simulink model "OSWEC_Hydraulic_PTO"  (R2020b)
settings: Solver=ode4  StartTime=0  StopTime=400  FixedStep=0.01  MaxStep=0.01  RelTol=1e-3  EnableMultiTasking=on
undefined symbols (not defined in the file or in its folder): body, constraint, geometry, hydroData, pto, PTOControl, ptoSim
libraries: WECSim_Lib_PTOSim x7, WECSim_Lib_Body_Elements x2, WECSim_Lib_Constraints x1, WECSim_Lib_Frames x1, pid_lib x1, WECSim_Lib_PTOs x1
settings Model: Creator=mlawson  LastModifiedBy=jleonqu
settings SolverCC: ZeroCrossControl=DisableAll  AlgebraicLoopSolver=LineSearch  AutoInsertRateTranBlk=on
settings DataIOCC: SaveFormat=Array  SaveOutput=off  SaveTime=off  ReturnWorkspaceOutputs=off
settings OptimizationCC: LifeSpan=inf  SimCompilerOptimization=on
settings DebuggingCC: UnderspecifiedInitializationDetection=Classic  MergeDetectMultiDrivingBlocksExec=none  SolverPrmCheckMsg=warning  AllowSymbolicDim=off  StateNameClashWarn=warning  SFUnexpectedBacktrackingDiag=warning  SFNoUnconditionalDefaultTransitionDiag=warning  ArithmeticOperatorsInVariantConditions=warning
settings HardwareCC: ProdBitPerPointer=32  ProdBitPerSizeT=32  ProdBitPerPtrDiffT=32  ProdLargestAtomicFloat=None  ProdIntDivRoundTo=Undefined  ProdEndianess=Unspecified  ProdWordSize=32  ProdHWDeviceType=32-bit Generic
settings ModelReferenceCC: PropagateSignalLabelsOutOfModel=off
settings SFSimCC: SimUseLocalCustomCode=off  CustomCodeUndefinedFunction=UseInterfaceOnly
settings RTWCC: RTWUseLocalCustomCode=off
settings CodeAppCC: StateflowObjectComments=on
settings GRTTargetCC: TargetLangStandard=C89/C90 (ANSI)
settings ConfigComp: CovMetricSettings=dw  CovSaveCumulativeToWorkspaceVar=on  CovSaveSingleToWorkspaceVar=on  CovExternalEMLEnable=off  CovSFcnEnable=off
settings SimscapeCC: SimscapeNormalizeSystem=off
settings ConfigurationSet: Description=SimMechanics 2G
settings ExplorerConfigSet: SimMechanicsOpenEditorOnUpdate=off  InternalSimMechanicsExplorerSettings="<ExplorerConfiguration><canonicalview>default</canonicalview><TilePanel><TileInfo><Tiles Columns=\"1\" Count=\"1\" Rows=\"1\"><Column Left=\"2\" Weight=\"1\"/><Column Left=\"1335\"/><Row Top=\"2\" Weight=\"1\"/><Row Top=\"911\"/><Tile Height=\"1\" Width=\"1\" X=\"0\" Y=\"0\"/></Tiles></TileInfo><SceneInfo><SceneViewer><BGColor><R>0.60000002384185791</R><G>0.60000002384185791</G><B>0.60000002384185791</B></BGColor><Camera><Position><X>365.37645888990272</X><Y>-369.82486814446582</Y><Z>359.64809521743916</Z></Position><Center><X>-6.7351450971904585</X><Y>2.2867358426280204</Y><Z>-12.463508769654169</Z></Center><Up><X>-0.40824829046386307</X><Y>0.40824829046386307</Y><Z>0.81649658092772615</Z></Up><Left>-57.820127362122818</Left><Right>57.820127362122818</Right><Bottom>-38.308817187253304</Bottom><Top>38.308817187253304</Top></Camera></SceneViewer></SceneInfo></TilePanel></ExplorerConfiguration>"

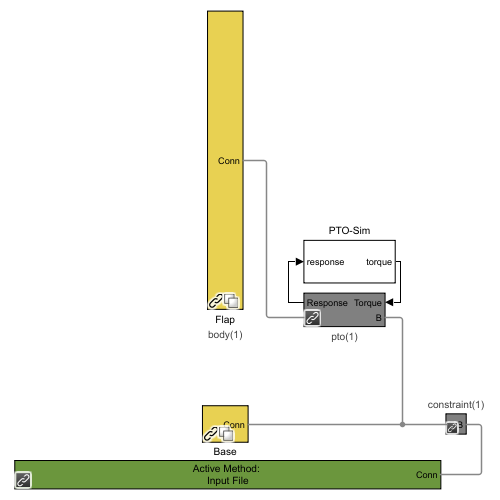
[thumbnail: Simulink's stored preview of the top-level diagram]
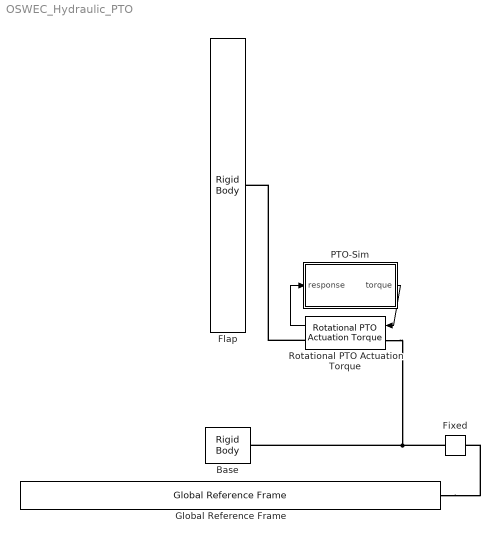
== system OSWEC_Hydraulic_PTO ==
  Base : WECSim_Lib_Body_Elements/Rigid Body  body=body(2)  h5File=hydroData/*.h5  geometryFile=geometry/*.stl  mass=0  inertia=0 0 0  inertiaProducts=0 0 0  nonHydro=0  nonlinearHydro=0  centerGravity=0 0 0  centerBuoyancy=0 0 0  dof=6  volume=0  displacement=0 0 0  axis=0 1 0  angle=0  option=0  cd=0 0 0  ca=0 0 0  area=0 0 0  VME=0  rgME=0 0 0  z=0 0 1
  Fixed : WECSim_Lib_Constraints/Fixed  constraint=constraint(1)  loc="0  0  0"  displacement=0 0 0  y=0 1 0  z=0 0 1  upperLimitSpecify=off  upperLimitBound=0  upperLimitTransitionRegionWidth=0  upperLimitStiffness=0  upperLimitDamping=0  lowerLimitSpecify=off  lowerLimitBound=0  lowerLimitTransitionRegionWidth=0  lowerLimitStiffness=0  lowerLimitDamping=0
      settings: AttributesFormatString=%<constraint>
  Flap : WECSim_Lib_Body_Elements/Rigid Body  body=body(1)  h5File=hydroData/*.h5  geometryFile=geometry/*.stl  mass=0  inertia=0 0 0  inertiaProducts=0 0 0  nonHydro=0  nonlinearHydro=0  centerGravity=0 0 0  centerBuoyancy=0 0 0  dof=6  volume=0  displacement=0 0 0  axis=0 1 0  angle=0  option=0  cd=0 0 0  ca=0 0 0  area=0 0 0  VME=0  rgME=0 0 0  z=0 0 1
  Global Reference Frame : WECSim_Lib_Frames/Global Reference Frame  waves=waves  simu=simu  InputMethod=Input File  InputFile=wecSimInputFile.m  mode=normal  explorer=off  solver=ode4  startTime=0  rampTime=100  endTime=400  dt=0.1  cicEndTime=60  stateSpace=0  WaveClass=regular  height=2.5  period=8  elevationFile=NOT DEFINED  spectrumFile=NOT DEFINED  direction=0  spread=1  spectrumType=NOT DEFINED  phaseSeed=0  option=EqualEnergy
  PTO-Sim : Subsystem
  Rotational PTO Actuation Torque : WECSim_Lib_PTOs/Rotational PTO Actuation Torque  pto=pto(1)  loc="0  0  0"  stiffness=0  damping=0  equilibriumPosition=0  pretension=0  displacement=0 0 0  y=0 1 0  z=0 0 1  upperLimitSpecify=off  upperLimitBound=0  upperLimitTransitionRegionWidth=0  upperLimitStiffness=0  upperLimitDamping=0  lowerLimitSpecify=off  lowerLimitBound=0  lowerLimitTransitionRegionWidth=0  lowerLimitStiffness=0  lowerLimitDamping=0
      settings: AttributesFormatString=%<pto>
  wires:
  Rotational PTO Actuation Torque/1 -> PTO-Sim/1(response)
  PTO-Sim/1(torque) -> Rotational PTO Actuation Torque/1
  connections:
  Global Reference Frame/RConn1 -- Fixed/LConn1
  Fixed/RConn1 -- Rotational PTO Actuation Torque/LConn1 -- Base/RConn1
  Rotational PTO Actuation Torque/RConn1 -- Flap/RConn1

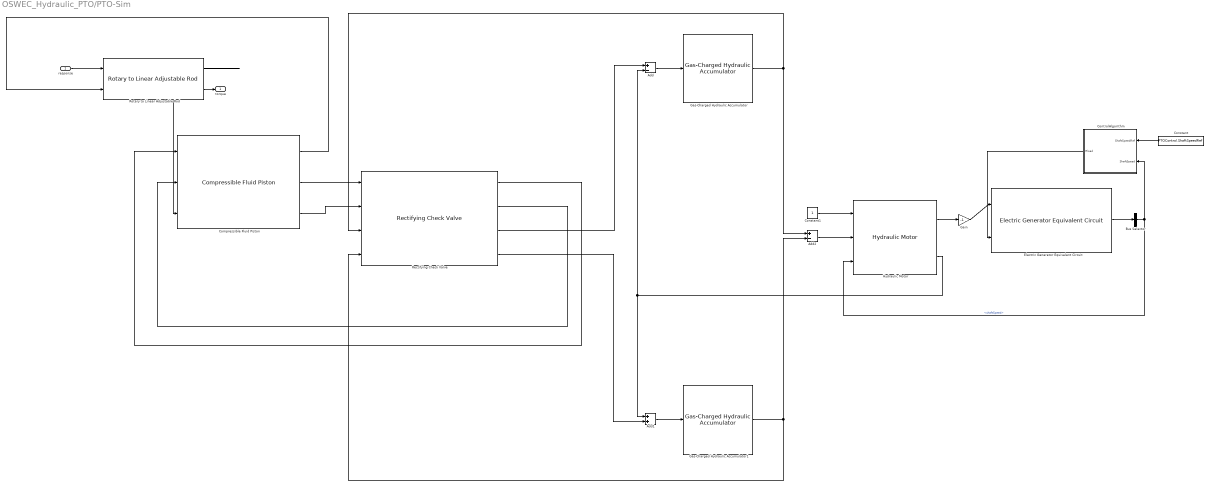
== system OSWEC_Hydraulic_PTO/PTO-Sim ==
  response : Inport
  Add : Sum  Inputs=+-
  Add1 : Sum
  Add2 : Sum  Inputs=+-
  Bus Selector : BusSelector  OutputSignals=shaftSpeed
  Compressible Fluid Piston : WECSim_Lib_PTOSim/Hydraulic/Compressible Fluid Piston  ptoSim=ptoSim(2)  Ap_A=0  Ap_B=0  pistonStroke=0  bulkModulus=0  xi_piston=0  pAi=0  pBi=0
  Constant : Constant  Value=PTOControl.ShaftSpeedRef
  Constant1 : Constant
  ControlAlgorithm : Subsystem
  Electric Generator Equivalent Circuit : WECSim_Lib_PTOSim/Electric/Electric Generator Equivalent Circuit  ptoSim=ptoSim(7)  Ra=0  La=0  Ke=0  bShaft=0  Jem=0
  Gain : Gain  Gain=-1
  Gas-Charged Hydraulic Accumulator : WECSim_Lib_PTOSim/Hydraulic/Gas-Charged Hydraulic Accumulator  ptoSim=ptoSim(4)  vI0=0  pIprecharge=0
  Gas-Charged Hydraulic Accumulator1 : WECSim_Lib_PTOSim/Hydraulic/Gas-Charged Hydraulic Accumulator  ptoSim=ptoSim(5)  vI0=0  pIprecharge=0
  Hydraulic Motor : WECSim_Lib_PTOSim/Hydraulic/Hydraulic Motor  ptoSim=ptoSim(6)  displacement=0  effModelVar=Analytical  effTableDeltaP=0  effTableShaftSpeed=0  effTableMechEff=0  effTableVolEff=0  wNominal=0  deltaPNominal=0  visNominal=0  densityNominal=0  effVolNom=0  torqueNoLoad=0  torqueVsPressure=0  rho=0  viscosity=0
  Rectifying Check Valve : WECSim_Lib_PTOSim/Hydraulic/Rectifying Check Valve  ptoSim=ptoSim(3)  Cd=0  Amax=0  Amin=0  pMin=0  pMax=0  rho=0  k1=0  k2=0
  Rotary to Linear Adjustable Rod : WECSim_Lib_PTOSim/Motion Conversion/Rotary to Linear Adjustable Rod  ptoSim=ptoSim(1)  crank=0  offset=0  rodInit=0
  torque : Outport  VectorParamsAs1DForOutWhenUnconnected=off
  wires:
  Hydraulic Motor/2 -> Add1/1, Add/2
  Add1/1 -> Gas-Charged Hydraulic Accumulator1/1
  Constant1/1 -> Hydraulic Motor/1
  Rectifying Check Valve/4 -> Add1/2
  Constant/1 -> ControlAlgorithm/1(ShaftSpeedRef)
  Hydraulic Motor/1 -> Gain/1
  ControlAlgorithm/1(Rload) -> Electric Generator Equivalent Circuit/2
  Add2/1 -> Hydraulic Motor/2
  Compressible Fluid Piston/2 -> Rectifying Check Valve/1
  Electric Generator Equivalent Circuit/1 -> Bus Selector/1
  Rectifying Check Valve/3 -> Add/1
  Bus Selector/1 -> Hydraulic Motor/3, ControlAlgorithm/2(ShaftSpeed)  "<shaftSpeed>"
  Rotary to Linear Adjustable Rod/2 -> torque/1
  Gas-Charged Hydraulic Accumulator1/1 -> Rectifying Check Valve/4, Add2/2
  Add/1 -> Gas-Charged Hydraulic Accumulator/1
  Gain/1 -> Electric Generator Equivalent Circuit/1
  Rotary to Linear Adjustable Rod/1 -> Compressible Fluid Piston/3
  Compressible Fluid Piston/3 -> Rectifying Check Valve/2
  Compressible Fluid Piston/1 -> Rotary to Linear Adjustable Rod/2
  Rectifying Check Valve/2 -> Compressible Fluid Piston/2
  Rectifying Check Valve/1 -> Compressible Fluid Piston/1
  response/1 -> Rotary to Linear Adjustable Rod/1
  Gas-Charged Hydraulic Accumulator/1 -> Rectifying Check Valve/3, Add2/1

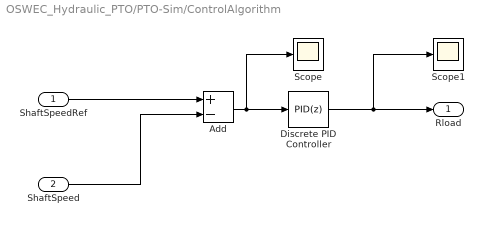
== system OSWEC_Hydraulic_PTO/PTO-Sim/ControlAlgorithm ==
  ShaftSpeedRef : Inport
  ShaftSpeed : Inport  Port=2
  Add : Sum  Inputs=+-
  Discrete PID Controller : pid_lib/PID Controller  Controller=PID  Form=Parallel  TimeDomain=Discrete-time  UseExternalTs=off  SampleTime=-1  IntegratorMethod=Forward Euler  ControllerParametersSource=internal  P=PTOControl.PG  I=PTOControl.IG  D=0  N=100  UseFilter=on  TunerSelectOption=Transfer Function Based (PID Tuner App)  InitialConditionSource=internal  InitialConditionForIntegrator=0  InitialConditionForFilter=0  DifferentiatorICPrevScaledInput=0  ExternalReset=none  TrackingMode=off  Kt=1  LimitOutput=off  SatLimitsSource=internal  UpperSaturationLimit=inf  LowerSaturationLimit=-inf  LinearizeAsGain=off  AntiWindupMode=none  Kb=1  POutMin=[]  POutMax=[]  IOutMin=[]  IOutMax=[]  DOutMin=[]  DOutMax=[]  NOutMin=[]  NOutMax=[]  SumOutMin=[]  SumOutMax=[]  SaturationOutMin=[]  SaturationOutMax=[]  PParamMin=[]  PParamMax=[]  IParamMin=[]  IParamMax=[]  DParamMin=[]  DParamMax=[]  NParamMin=[]  NParamMax=[]  KbParamMin=[]  KbParamMax=[]  KtParamMin=[]  KtParamMax=[]  KbOutMin=[]  KbOutMax=[]  KtOutMin=[]  KtOutMax=[]  IntegratorOutMin=[]  IntegratorOutMax=[]  FilterOutMin=[]  FilterOutMax=[]  SumI1OutMin=[]  SumI1OutMax=[]  SumI2OutMin=[]  SumI2OutMax=[]  SumI3OutMin=[]  SumI3OutMax=[]  SumI4OutMin=[]  SumI4OutMax=[]  SumDOutMin=[]  SumDOutMax=[]  DifferentiatorOutMin=[]  DifferentiatorOutMax=[]  FilterDiffOutCoefMin=[]  FilterDiffOutCoefMax=[]  ReciprocalOutMin=[]  ReciprocalOutMax=[]  SumDenOutMin=[]  SumDenOutMax=[]  SumNumOutMin=[]  SumNumOutMax=[]  DivideOutMin=[]  DivideOutMax=[]  UdiffTsProdOutMin=[]  UdiffTsProdOutMax=[]  NTsProdOutMin=[]  NTsProdOutMax=[]  UintegralTsProdOutMin=[]  UintegralTsProdOutMax=[]  UngainTsProdOutMin=[]  UngainTsProdOutMax=[]  IntegratorContinuousStateAttributes=''  IntegratorStateMustResolveToSignalObject=off  IntegratorRTWStateStorageClass=Auto  FilterContinuousStateAttributes=''  FilterStateMustResolveToSignalObject=off  FilterRTWStateStorageClass=Auto  ParallelPVariant=InternalParameters  IdealPVariant=Disabled  IVariant=InternalParameters  DVariant=InternalParameters  IntegratorVariant=Discrete  SatVariant=Disabled  AWVariant=Passthrough  PCopyVariant=Disabled  TRVariant=Disabled  FdbkBlocksVariant=Forward  IdealPFdbkVariant=Disabled  SatFdbkVariant=Disabled  DerivativeFilterVariant=ForwardEulerFilter  NVariant=InternalParameters  NCopyVariant=Disabled  FilterICVariant=InternalICsFilter  IntegratorICVariant=InternalICs  ExternalResetVariant=Disabled  TRSumVariant=Passthrough  SumFdbkVariant=Disabled  SumVariant=Sum_PID  TsampFilterVariant=InternalTs  TsampNgainVariant=Passthrough  TsampIntegralVariant=Passthrough  ExternalSaturationOutDataTypeStr=Inherit: Same as second input
  Scope : Scope
  Scope1 : Scope
  Rload : Outport
  wires:
  Discrete PID Controller/1 -> Scope1/1, Rload/1
  Add/1 -> Scope/1, Discrete PID Controller/1
  ShaftSpeedRef/1 -> Add/1
  ShaftSpeed/1 -> Add/2
